simulink model "ASM_Traffic_new"  (R2024a)
settings: Solver=ode1  StartTime=SIM.tstart.v  StopTime=SIM.tend.v  FixedStep=SIM.StepSize.v  RelTol=1e-3
PostLoadFcn:
  | if any(exist('dsrtsu_mdlpostloadfcn', 'file') ~= 0), dsrtsu_mdlpostloadfcn('Execute', bdroot); end
  | try, asm_mdl_postloadfcn(bdroot, 'UpdateModel', 3600); catch, disp(lasterr); end,
InitFcn:
  | , if any(exist('rtifpga_mdlclblib', 'file') ~= 0), rtifpga_mdlclblib('Init', bdroot); end,
  | , if any(exist('dsmpb_private', 'file') ~= 0), dsmpb_private('dsmpb_mdlclblib', 'Init', bdroot); end,
undefined symbols (not defined in the file): _to_, a0b2, ASM_BrakeHydraulics_DemoSystems, ASM_VehicleDynamics_DemoSystems, b98103fe8ad365046cd0, BrakeCircuit, CPT, Crankshaft, DiscIntNeverNeededParam, dsmsi, FinalDriveAssembly, MDL, ModeSignals, Pos_BrakePedal_Maneuver, rad, RefSignals, s_to_rpm, SIM, SoftECU, Suspension, Tire, Transmission
libraries: ASM_Traffic_lib x135, simulink x100, ASM_Utils_lib x77, ASM_VehicleDynamics_lib x70, ASM_Environment_lib x22, dsmpblib x20, dsmsilib x15, MDLD_Utils_lib x10, ASM_BrakeHydraulics_lib x3
(part 4 of 63)

== system ASM_Traffic_new/Environment/Interface_In ==
  note: Environment Traffic
  In : Inport
  Bus Creator1 : BusCreator  Inputs=1
  Bus Selector1 : BusSelector  OutputSignals=Environment.Plant.Sw_ModelPortBlocks[0Disabled|1Enabled],Environment.Plant.Sw_ModelDeskPlottingInterface[0Disabled|1Enabled],VehicleDynamics.Plant.Angle_SteeringWheel[deg],VehicleDynamics.Plant.Angle_SteeringWheel_dt[deg|s],VehicleDynamics.Plant.Trq_SteeringWheel[Nm],VehicleDynamics.Plant.r_Dyn_Tire[FL;FR;RL;RR][m],VehicleDynamics.Plant.Coef_RollingRes[FL;FR;RL;RR][],VehicleDynamics.Plant.CorneringStiffness[FL;FR;RL;RR][N],VehicleDynamics.Plant.Pos_Vehicle_CoorSys_E[x;y;z][m],VehicleDynamics.Plant.Angle_Vehicle_CoorSys_E[x;y;z][deg],VehicleDynamics.Plant.s_Vehicle[m],VehicleDynamics.Plant.v_x_Vehicle_CoG[km|h],VehicleDynamics.Plant.v_y_Vehicle_CoG[km|h],VehicleDynamics.Plant.RollRate_Vehicle_CoG[deg|s],VehicleDynamics.Plant.YawRate_Vehicle_CoG[deg|s],VehicleDynamics.Plant.a_y_Vehicle_CoG[m|s2],VehicleDynamics.Plant.RotationMatrix_V_to_E[1x9],VehicleDynamics.Plant.Const_r_unloaded_Tire_Mean[m],VehicleDynamics.Plant.Coef_RollingRes_Mean[],DomainControl.DriverAssistance.Control.AEB[0|1],DomainControl.DriverAssistance.Control.FCW[0|1],Driver.Plant.Pos_AccPedal[%],Driver.Plant.Pos_BrakePedal[%],Driver.Plant.Pos_ClutchPedal[%],Drivetrain.Plant.Gear[],Driver.Plant.SelectorLever[-3T|-2P|-1R|0N|1D],Driver.Plant.s_Preview[m],Driver.Plant.Angle_SteeringWheel[deg],Driver.Plant.t_Preview_vRef_Driver[s],Drivetrain.Plant.Type_Engine_1[0Unkown|1Other|2Otto|3Diesel|4Electric],Drivetrain.Plant.Trq_Engine_1[Nm],Drivetrain.Plant.n_Engine_1[rpm],Drivetrain.Plant.Type_Engine_2[0Unkown|1Other|2Otto|3Diesel|4Electric],Drivetrain.Plant.Trq_Engine_2[Nm],Drivetrain.Plant.n_Engine_2[rpm],VehicleDynamics.Plant.m_TotalVehicle[kg],DomainControl.StartSystem.Control.State_StartButton[-2|-1|0|1|2|3],DomainControl.DriverAssistance.Control.ACC_State[1OFF|2Standby|3ON],DomainControl.DriverAssistance.Control.Driver_Override_ACC_Active[0Off|1On],DomainControl.DriverAssistance.Control.Driver_Override_ACC_Reason[0NoOverride|1BrakePedal|2AccPedal],VehicleDynamics.Plant.omega_Wheel[rad|s],VehicleDynamics.Plant.Slip_x_Wheel[],VehicleDynamics.Plant.Pos_CP_FL_CoorSys_E[x;y][m],VehicleDynamics.Plant.Pos_CP_FR_CoorSys_E[x;y][m],VehicleDynamics.Plant.Pos_CP_RL_CoorSys_E[x;y][m],VehicleDynamics.Plant.Pos_CP_RL2_CoorSys_E[x;y][m],VehicleDynamics.Plant.Pos_CP_RR_CoorSys_E[x;y][m],VehicleDynamics.Plant.Pos_CP_RR2_CoorSys_E[x;y][m],VehicleDynamics.Plant.Pos_CP_R2L_CoorSys_E[x;y][m],VehicleDynamics.Plant.Pos_CP_R2L2_CoorSys_E[x;y][m],VehicleDynamics.Plant.Pos_CP_R2R_CoorSys_E[x;y][m],VehicleDynamics.Plant.Pos_CP_R2R2_CoorSys_E[x;y][m],Drivetrain.Plant.Mode_Transmission[1Manual|2Automatic],Drivetrain.Plant.Mode_Drivetrain[1|2|3|4|5],VehicleDynamics.Plant.Sw_MasterBrakeCylinder_Mode[1linear|2physical|3Booster],VehicleDynamics.Plant.Active_CP_VehDyn[],VehicleDynamics.Plant.Pos_CP_Front_CoorSys_E[x;y][m],VehicleDynamics.Plant.Pos_CP_Rear_CoorSys_E[x;y][m]
  ModelSignals : Subsystem
  Pos_CP_FL2_Trailer_CoorSys_E[x;y][m] : Constant  Value=[0;0]
  Pos_CP_FL_Trailer_CoorSys_E[x;y][m] : Constant  Value=[0;0]
  Pos_CP_FR2_Trailer_CoorSys_E[x;y][m] : Constant  Value=[0;0]
  Pos_CP_FR_Trailer_CoorSys_E[x;y][m] : Constant  Value=[0;0]
  Pos_CP_R2L2_Trailer_CoorSys_E[x;y][m] : Constant  Value=[0;0]
  Pos_CP_R2L_Trailer_CoorSys_E[x;y][m] : Constant  Value=[0;0]
  Pos_CP_R2R2_Trailer_CoorSys_E[x;y][m] : Constant  Value=[0;0]
  Pos_CP_R2R_Trailer_CoorSys_E[x;y][m] : Constant  Value=[0;0]
  Pos_CP_RL2_Trailer_CoorSys_E[x;y][m] : Constant  Value=[0;0]
  Pos_CP_RL_Trailer_CoorSys_E[x;y][m] : Constant  Value=[0;0]
  Pos_CP_RR2_Trailer_CoorSys_E[x;y][m] : Constant  Value=[0;0]
  Pos_CP_RR_Trailer_CoorSys_E[x;y][m] : Constant  Value=[0;0]
  Out : Outport  VectorParamsAs1DForOutWhenUnconnected=off
  wires:
  Bus Creator1/1 -> Out/1  "Interface_In"
  ModelSignals/1(Out) -> Bus Creator1/1
  Pos_CP_FL_Trailer_CoorSys_E[x;y][m]/1 -> ModelSignals/57(Pos_CP_FL_Trailer_CoorSys_E[x;y][m])
  Pos_CP_FL2_Trailer_CoorSys_E[x;y][m]/1 -> ModelSignals/58(Pos_CP_FL2_Trailer_CoorSys_E[x;y][m])
  Pos_CP_FR_Trailer_CoorSys_E[x;y][m]/1 -> ModelSignals/59(Pos_CP_FR_Trailer_CoorSys_E[x;y][m])
  Pos_CP_FR2_Trailer_CoorSys_E[x;y][m]/1 -> ModelSignals/60(Pos_CP_FR2_Trailer_CoorSys_E[x;y][m])
  Pos_CP_RL_Trailer_CoorSys_E[x;y][m]/1 -> ModelSignals/61(Pos_CP_RL_Trailer_CoorSys_E[x;y][m])
  Pos_CP_RL2_Trailer_CoorSys_E[x;y][m]/1 -> ModelSignals/62(Pos_CP_RL2_Trailer_CoorSys_E[x;y][m])
  Pos_CP_RR_Trailer_CoorSys_E[x;y][m]/1 -> ModelSignals/63(Pos_CP_RR_Trailer_CoorSys_E[x;y][m])
  Pos_CP_RR2_Trailer_CoorSys_E[x;y][m]/1 -> ModelSignals/64(Pos_CP_RR2_Trailer_CoorSys_E[x;y][m])
  Pos_CP_R2L_Trailer_CoorSys_E[x;y][m]/1 -> ModelSignals/65(Pos_CP_R2L_Trailer_CoorSys_E[x;y][m])
  Pos_CP_R2L2_Trailer_CoorSys_E[x;y][m]/1 -> ModelSignals/66(Pos_CP_R2L2_Trailer_CoorSys_E[x;y][m])
  Pos_CP_R2R_Trailer_CoorSys_E[x;y][m]/1 -> ModelSignals/67(Pos_CP_R2R_Trailer_CoorSys_E[x;y][m])
  Pos_CP_R2R2_Trailer_CoorSys_E[x;y][m]/1 -> ModelSignals/68(Pos_CP_R2R2_Trailer_CoorSys_E[x;y][m])
  Bus Selector1/1 -> ModelSignals/1(Sw_ModelPortBlocks[0Disabled|1Enabled])  "<Sw_ModelPortBlocks[0Disabled|1Enabled]>"
  Bus Selector1/2 -> ModelSignals/2(Sw_ModelDeskPlottingInterface[0Disabled|1Enabled])  "<Sw_ModelDeskPlottingInterface[0Disabled|1Enabled]>"
  Bus Selector1/3 -> ModelSignals/3(Angle_SteeringWheel_SteeringSystem[deg])  "<Angle_SteeringWheel[deg]>"
  Bus Selector1/4 -> ModelSignals/4(Angle_SteeringWheel_dt_SteeringSystem[deg|s])  "<Angle_SteeringWheel_dt[deg|s]>"
  Bus Selector1/5 -> ModelSignals/5(Trq_SteeringWheel_SteeringSystem[Nm])  "<Trq_SteeringWheel[Nm]>"
  Bus Selector1/6 -> ModelSignals/6(r_Dyn_Tire[FL;FR;RL;RR][m])  "<r_Dyn_Tire[FL;FR;RL;RR][m]>"
  Bus Selector1/7 -> ModelSignals/7(Coef_RollingRes[FL;FR;RL;RR][])  "<Coef_RollingRes[FL;FR;RL;RR][]>"
  Bus Selector1/8 -> ModelSignals/8(CorneringStiffness[FL;FR;RL;RR][N])  "<CorneringStiffness[FL;FR;RL;RR][N]>"
  Bus Selector1/9 -> ModelSignals/9(Pos_Vehicle_CoorSys_E[x;y;z][m])  "<Pos_Vehicle_CoorSys_E[x;y;z][m]>"
  Bus Selector1/10 -> ModelSignals/10(Angle_Vehicle_CoorSys_E[x;y;z][deg])  "<Angle_Vehicle_CoorSys_E[x;y;z][deg]>"
  Bus Selector1/11 -> ModelSignals/11(s_Vehicle[m])  "<s_Vehicle[m]>"
  Bus Selector1/12 -> ModelSignals/12(v_x_Vehicle_CoG[km|h])  "<v_x_Vehicle_CoG[km|h]>"
  Bus Selector1/13 -> ModelSignals/13(v_y_Vehicle_CoG[km|h])  "<v_y_Vehicle_CoG[km|h]>"
  Bus Selector1/14 -> ModelSignals/14(RollRate_Vehicle_CoG[deg|s])  "<RollRate_Vehicle_CoG[deg|s]>"
  Bus Selector1/15 -> ModelSignals/15(YawRate_Vehicle_CoG[deg|s])  "<YawRate_Vehicle_CoG[deg|s]>"
  Bus Selector1/16 -> ModelSignals/16(a_y_Vehicle_CoG[m|s2])  "<a_y_Vehicle_CoG[m|s2]>"
  Bus Selector1/17 -> ModelSignals/17(RotationMatrix_V_to_E[1x9])  "<RotationMatrix_V_to_E[1x9]>"
  Bus Selector1/18 -> ModelSignals/18(Const_r_unloaded_Tire_Mean[m])  "<Const_r_unloaded_Tire_Mean[m]>"
  Bus Selector1/19 -> ModelSignals/19(Coef_RollingRes_Mean[])  "<Coef_RollingRes_Mean[]>"
  Bus Selector1/20 -> ModelSignals/20(AEB[0|1])  "<AEB[0|1]>"
  Bus Selector1/21 -> ModelSignals/21(FCW[0|1])  "<FCW[0|1]>"
  Bus Selector1/22 -> ModelSignals/22(Pos_AccPedal[%])  "<Pos_AccPedal[%]>"
  Bus Selector1/23 -> ModelSignals/23(Pos_BrakePedal[%])  "<Pos_BrakePedal[%]>"
  Bus Selector1/24 -> ModelSignals/24(Pos_ClutchPedal[%])  "<Pos_ClutchPedal[%]>"
  Bus Selector1/25 -> ModelSignals/25(Gear[])  "<Gear[]>"
  Bus Selector1/26 -> ModelSignals/26(SelectorLever[-3T|-2P|-1R|0N|1D])  "<SelectorLever[-3T|-2P|-1R|0N|1D]>"
  Bus Selector1/27 -> ModelSignals/27(s_Preview[m])  "<s_Preview[m]>"
  Bus Selector1/28 -> ModelSignals/28(Angle_SteeringWheel[deg])  "<Angle_SteeringWheel[deg]>"
  Bus Selector1/29 -> ModelSignals/29(t_Preview_vRef_Driver[s])  "<t_Preview_vRef_Driver[s]>"
  Bus Selector1/30 -> ModelSignals/30(Type_Engine_1[0Unkown|1Other|2Otto|3Diesel|4Electric])  "<Type_Engine_1[0Unkown|1Other|2Otto|3Diesel|4Electric]>"
  Bus Selector1/31 -> ModelSignals/31(Trq_Engine_1[Nm])  "<Trq_Engine_1[Nm]>"
  Bus Selector1/32 -> ModelSignals/32(n_Engine_1[rpm])  "<n_Engine_1[rpm]>"
  Bus Selector1/33 -> ModelSignals/33(Type_Engine_2[0Unkown|1Other|2Otto|3Diesel|4Electric])  "<Type_Engine_2[0Unkown|1Other|2Otto|3Diesel|4Electric]>"
  Bus Selector1/34 -> ModelSignals/34(Trq_Engine_2[Nm])  "<Trq_Engine_2[Nm]>"
  Bus Selector1/35 -> ModelSignals/35(n_Engine_2[rpm])  "<n_Engine_2[rpm]>"
  Bus Selector1/36 -> ModelSignals/36(m_TotalVehicle[kg])  "<m_TotalVehicle[kg]>"
  Bus Selector1/37 -> ModelSignals/37(State_StartButton[-2|-1|0|1|2|3])  "<State_StartButton[-2|-1|0|1|2|3]>"
  Bus Selector1/38 -> ModelSignals/38(ACC_State[1OFF|2Standby|3ON])  "<ACC_State[1OFF|2Standby|3ON]>"
  Bus Selector1/39 -> ModelSignals/39(Driver_Override_ACC_Active[0Off|1On])  "<Driver_Override_ACC_Active[0Off|1On]>"
  Bus Selector1/40 -> ModelSignals/40(Driver_Override_ACC_Reason[0NoOverride|1BrakePedal|2AccPedal])  "<Driver_Override_ACC_Reason[0NoOverride|1BrakePedal|2AccPedal]>"
  Bus Selector1/41 -> ModelSignals/41(omega_Wheel[rad|s])  "<omega_Wheel[rad|s]>"
  Bus Selector1/42 -> ModelSignals/42(Slip_x_Wheel[])  "<Slip_x_Wheel[]>"
  Bus Selector1/43 -> ModelSignals/43(Pos_CP_FL_CoorSys_E[x;y][m])  "<Pos_CP_FL_CoorSys_E[x;y][m]>"
  Bus Selector1/44 -> ModelSignals/44(Pos_CP_FR_CoorSys_E[x;y][m])  "<Pos_CP_FR_CoorSys_E[x;y][m]>"
  Bus Selector1/45 -> ModelSignals/45(Pos_CP_RL_CoorSys_E[x;y][m])  "<Pos_CP_RL_CoorSys_E[x;y][m]>"
  Bus Selector1/46 -> ModelSignals/46(Pos_CP_RL2_CoorSys_E[x;y][m])  "<Pos_CP_RL2_CoorSys_E[x;y][m]>"
  Bus Selector1/47 -> ModelSignals/47(Pos_CP_RR_CoorSys_E[x;y][m])  "<Pos_CP_RR_CoorSys_E[x;y][m]>"
  Bus Selector1/48 -> ModelSignals/48(Pos_CP_RR2_CoorSys_E[x;y][m])  "<Pos_CP_RR2_CoorSys_E[x;y][m]>"
  Bus Selector1/49 -> ModelSignals/49(Pos_CP_R2L_CoorSys_E[x;y][m])  "<Pos_CP_R2L_CoorSys_E[x;y][m]>"
  Bus Selector1/50 -> ModelSignals/50(Pos_CP_R2L2_CoorSys_E[x;y][m])  "<Pos_CP_R2L2_CoorSys_E[x;y][m]>"
  Bus Selector1/51 -> ModelSignals/51(Pos_CP_R2R_CoorSys_E[x;y][m])  "<Pos_CP_R2R_CoorSys_E[x;y][m]>"
  Bus Selector1/52 -> ModelSignals/52(Pos_CP_R2R2_CoorSys_E[x;y][m])  "<Pos_CP_R2R2_CoorSys_E[x;y][m]>"
  Bus Selector1/53 -> ModelSignals/53(Mode_Transmission[1Manual|2Automatic])  "<Mode_Transmission[1Manual|2Automatic]>"
  Bus Selector1/54 -> ModelSignals/54(Mode_Drivetrain[1|2|3|4|5])  "<Mode_Drivetrain[1|2|3|4|5]>"
  Bus Selector1/55 -> ModelSignals/55(Sw_MasterBrakeCylinder_Mode[1linear|2physical|3Booster])  "<Sw_MasterBrakeCylinder_Mode[1linear|2physical|3Booster]>"
  Bus Selector1/56 -> ModelSignals/56(Active_CP_VehDyn_Trailer[])  "<Active_CP_VehDyn[]>"
  Bus Selector1/57 -> ModelSignals/69(Pos_CP_Front_CoorSys_E[x;y][m])  "<Pos_CP_Front_CoorSys_E[x;y][m]>"
  Bus Selector1/58 -> ModelSignals/70(Pos_CP_Rear_CoorSys_E[x;y][m])  "<Pos_CP_Rear_CoorSys_E[x;y][m]>"
  In/1 -> Bus Selector1/1

== system ASM_Traffic_new/Environment/Interface_Out ==
  note: Environment Traffic
  In : Inport
  Activate_DCLink[0Off|1On] : Constant  Value=0
  Animation : Subsystem
  Bus Creator1 : BusCreator  Inputs=2
  Bus Selector1 : BusSelector  OutputSignals=FellowVehicleLights,FellowVehicleDoors  OutputAsBus=on
  Bus Selector{10..12,14,16..18} (7 alike) : BusSelector  OutputSignals=Parameters.Pos_Sensor_Apex_CoorSys_V[x;y;z][m],Parameters.Angle_z_Orientation_Sensor_CoorSys_V[deg],SensorOutput.Angle_Hor_Rel[deg],SensorOutput.Distance[m],Parameters.Num_SensorRays_Used[],Parameters.Angle_ScopeZone_Horizontal[deg]  OutputAsBus=on
  Bus Selector13 : BusSelector  OutputSignals=Line_Sensor_1.Pos_Road_Lane_Animation_CoorSys_E,Line_Sensor_1.Pos_Road_Shape_Line_Animation_CoorSys_E,Line_Sensor_1.Pos_Road_Shape_ContObj_Animation_CoorSys_E,Line_Sensor_1.Pos_Junction_Border_Animation_CoorSys_E,Line_Sensor_1.Pos_Junction_Shape_Line_Animation_CoorSys_E,Line_Sensor_1.Pos_Junction_Shape_ContObj_Animation_CoorSys_E  OutputAsBus=on
  Bus Selector19 : BusSelector  OutputSignals=Sensor_Front_1.SensorOutput[].Traffic_Sign_Valid[0|1],Sensor_Front_1.SensorOutput[].Pos_CoorSys_E[x;y;z][m]  OutputAsBus=on
  Bus Selector20 : BusSelector  OutputSignals=SensorOutput.Pos_Object_NearestPnt_E[x;y;z][m],Info.Flag_Object_In_Scope[0Out|1In],SensorOutput.Flag_NearestPnt_Occluded[-1|0|1]  OutputAsBus=on
  Bus Selector21 : BusSelector  OutputSignals=SensorOutput.Pos_Object_NearestPnt_E[x;y;z][m],Info.Flag_Object_In_Scope[0Out|1In],SensorOutput.Flag_NearestPnt_Occluded[-1|0|1]  OutputAsBus=on
  Bus Selector22 : BusSelector  OutputSignals=ID[],Pos_ObjectPoint_CoorSys_E[x;y;z][m]  OutputAsBus=on
  Bus Selector23 : BusSelector  OutputSignals=ID[],Pos_CoorSys_E[x;y;z][m]  OutputAsBus=on
  Bus Selector24 : BusSelector  OutputSignals=ID[],Pos_ObjectPoint_CoorSys_E[x;y;z][m]  OutputAsBus=on
  Bus Selector25 : BusSelector  OutputSignals=ID[],Pos_ObjectPoint_CoorSys_E[x;y;z][m]  OutputAsBus=on
  Bus Selector26 : BusSelector  OutputSignals=ID[],Pos_CoorSys_E[x;y;z][m]  OutputAsBus=on
  Bus Selector27 : BusSelector  OutputSignals=ID[],Pos_CoorSys_E[x;y;z][m]  OutputAsBus=on
  Bus Selector28 : BusSelector  OutputSignals=SensorOutput.Pos_Object_NearestPnt_E[x;y;z][m],Info.Flag_Object_In_Scope[0Out|1In],SensorOutput.Flag_NearestPnt_Occluded[-1|0|1]  OutputAsBus=on
  Bus Selector3 : BusSelector  OutputSignals=Maneuver.UserInterface.Enable_External_Interfaces.Sw_AnimationInterface[0Disabled|1Enabled],Road.Plant.Road_ASMVeh.s_Veh_Road[m],Road.Plant.LaneSensor_Dynamic.Sensor_Output.CurrentLane.LeftSide.Pos_Left[x;y;z][m],Road.Plant.LaneSensor_Dynamic.Sensor_Output.CurrentLane.LeftSide.Yaw_Angle_Left[deg],Road.Plant.LaneSensor_Dynamic.Sensor_Output.CurrentLane.LeftSide.MarkerType_Left[],Road.Plant.LaneSensor_Dynamic.Sensor_Output.CurrentLane.RightSide.Pos_Right[x;y;z][m],Road.Plant.LaneSensor_Dynamic.Sensor_Output.CurrentLane.RightSide.Yaw_Angle_Right[deg],Road.Plant.LaneSensor_Dynamic.Sensor_Output.Lanes_Right.MarkerType_Right[],Road.Plant.Road_Info.Network_Item_Type_Veh[],Road.Plant.LaneSensor_Dynamic.Sensor_Output.Measurement_Points.Distance_MeasPnt_Marker_Left[m],Road.Plant.LaneSensor_Dynamic.Sensor_Output.Measurement_Points.Distance_MeasPnt_Marker_Right[m],Road.Plant.LaneSensor_Dynamic.Sensor_Output.Measurement_Points.Velocity_MeasPnt_Marker_Left[m|s],Road.Plant.LaneSensor_Dynamic.Sensor_Output.Measurement_Points.Velocity_MeasPnt_Marker_Right[m|s],Road.UserInterface.Objects_DataStreams[],Maneuver.Plant.ManeuverScheduler.Info.ManeuverTime[s],Maneuver.Plant.ManeuverScheduler.Info.ManeuverState[],Maneuver.UserInterface.ManualControl.VehicleLights.Sw_ManualControl_Lights[1Maneuver|2Manual],Maneuver.UserInterface.ManualControl.VehicleLights.Sw_BrakeLight[0Off|1On],Maneuver.UserInterface.ManualControl.VehicleLights.Sw_TurnLights[0Off|1Left|2Right|3Both],Maneuver.Plant.UserSignals_Customized.ASM_Vehicle_TurnLights[],Traffic.Plant.Traffic_Signals_toEnvironment.Pos_Fellows_MainPnt_CoorSys_E[x;y;z][m],Traffic.Plant.Traffic_Signals_toEnvironment.Angle_Fellows[x;y;z][deg],Traffic.Plant.Traffic_Signals_toEnvironment.Flag_FellowUsed[0|1],Traffic.Plant.Traffic_Signals_toEnvironment.v_Fellows_Ref_Scheduler[km|h],Traffic.Plant.Traffic_Signals_toEnvironment.a_Fellows_Ref_Scheduler[m|s2],Traffic.Plant.Traffic_Signals_toEnvironment.v_Fellows[km|h],Traffic.Plant.Traffic_Signals_toEnvironment.UserSignals_Customized,Traffic.UserInterface,Sensors.Plant.Object_Sensor_3D.Boundingboxes_DetectedObjects,Sensors.Plant.Object_Sensor_3D.Sensor_1_Front_Long,Sensors.Plant.Object_Sensor_3D.Sensor_2_Front_Mid,Sensors.Plant.Object_Sensor_3D.Sensor_3_Rear,Sensors.Plant.Object_Sensor_2D.Sensor_1_Front,Sensors.Plant.Object_Sensor_2D.Sensor_2_Front_Left,Sensors.Plant.Object_Sensor_2D.Sensor_3_Left,Sensors.Plant.Object_Sensor_2D.Sensor_4_Rear_Left,Sensors.Plant.Object_Sensor_2D.Sensor_5_Front_Right,Sensors.Plant.Object_Sensor_2D.Sensor_6_Right,Sensors.Plant.Object_Sensor_2D.Sensor_7_Rear_Right,Sensors.Plant.TrafficSign_Sensor_Dyn,Sensors.Plant.Line_Sensor,Sensors.Plant.Object_Sensor_3D.Sensor_1_Front_Long.RadarEffects,Sensors.Plant.Object_Sensor_3D.Sensor_2_Front_Mid.RadarEffects,Sensors.Plant.Object_Sensor_3D.Sensor_3_Rear.RadarEffects,Sensors.Plant.Object_Sensor_3D.Sensor_1_Front_Long.CustomPoints,Sensors.Plant.Object_Sensor_3D.Sensor_2_Front_Mid.CustomPoints,Sensors.Plant.Object_Sensor_3D.Sensor_3_Rear.CustomPoints,Maneuver.Plant.UserSignals_Customized.Mnv_DoorFL[],Maneuver.Plant.UserSignals_Customized.Mnv_DoorFR[],Maneuver.Plant.UserSignals_Customized.Mnv_DoorRL[],Maneuver.Plant.UserSignals_Customized.Mnv_DoorRR[],Maneuver.Plant.UserSignals_Customized.Mnv_Hood[],Maneuver.Plant.UserSignals_Customized.Mnv_Trunk[],Maneuver.UserInterface.ManualControl.Doors.Sw_ManualControl_Doors[1Maneuver|2Manual],Maneuver.UserInterface.ManualControl.Doors.Sw_DoorFL[0Closed_1Open],Maneuver.UserInterface.ManualControl.Doors.Sw_DoorFR[0Closed_1Open],Maneuver.UserInterface.ManualControl.Doors.Sw_DoorRL[0Closed_1Open],Maneuver.UserInterface.ManualControl.Doors.Sw_DoorRR[0Closed_1Open],Maneuver.UserInterface.ManualControl.Doors.Sw_Hood[0Closed_1Open],Maneuver.UserInterface.ManualControl.Doors.Sw_Trunk[0Closed_1Open]
  Bus Selector8 : BusSelector  OutputSignals=Maneuver.Plant.ManeuverScheduler.RefSignals.Pos_AccPedal_Maneuver[%],Maneuver.Plant.ManeuverScheduler.RefSignals.Pos_BrakePedal_Maneuver[%],Maneuver.Plant.ManeuverScheduler.RefSignals.Pos_ClutchPedal_Maneuver[%],Maneuver.Plant.ManeuverScheduler.RefSignals.Gear_Maneuver[],Maneuver.Plant.ManeuverScheduler.RefSignals.Angle_SteeringWheel_Maneuver[deg],Maneuver.Plant.ManeuverScheduler.RefSignals.SelectorLever_Maneuver[],Maneuver.Plant.Sw_TipShift[-1Down|0Off|1Up],Maneuver.Plant.Testbench.n_Engine_Set[rpm],Maneuver.Plant.Testbench.EngOpNum[],Maneuver.Plant.StartButton.Sw_StartButton[0Off|1On],Maneuver.Plant.ManeuverScheduler.RefSignals.v_Vehicle_Ref_Maneuver[m|s],Maneuver.Plant.ManeuverScheduler.RefSignals.v_Vehicle_Ref_Preview_Maneuver[m|s],Maneuver.Plant.ParkingBrake.Sw_ParkingBrake[0Off|1On],Maneuver.Plant.ManeuverScheduler.Parameters.a_x_Max[m|s2],Maneuver.Plant.ManeuverScheduler.Parameters.a_x_Brake_Threshold[m|s2],Maneuver.Plant.ManeuverScheduler.Parameters.a_y_Max[m|s2],Maneuver.Plant.ManeuverScheduler.Parameters.Gear_Max[],Maneuver.Plant.VehicleInitStates.Enable_v_Init[0|1],Traffic.Plant.Traffic_Signals_toEnvironment.a_x_Vehicle_Ref[m|s2],Maneuver.Plant.ManeuverScheduler.Parameters.Width_Deadzone_LatCtrl[m],Road.Plant.Road_ASMVeh.Pos_x_Ref_Veh_Road[m],Road.Plant.Road_ASMVeh.Pos_y_Ref_Veh_Road[m],Maneuver.Plant.ManeuverScheduler.MdlControl.Reset_VehicleStates[0|1],Maneuver.Plant.UserSignals_Customized.ECU_Commands[],Maneuver.Plant.VehicleInitStates.q_dt_Vehicle_Init[6x1],Maneuver.Plant.ManeuverScheduler.RefSignals.Trq_Steering_Maneuver[Nm],Maneuver.Plant.ManeuverScheduler.RefSignals.Sw_SteeringMode_Maneuver[1Angle|2Trq],Maneuver.Plant.ManeuverScheduler.InitialVehStates.s_Vehicle_Init[m],Maneuver.Plant.ManeuverScheduler.InitialVehStates.Route_Direction_Init[],Maneuver.Plant.StartButton.State_StartButton[-1PowerOff|0Acc|1PowerOn|2StarterOn],Road.Plant.Ambient.T_Ambient[degC],Road.Plant.Ambient.p_Ambient[Pa],Road.Plant.Road_ContactPoints.Pos_z_CP[:][m],Road.Plant.Road_ContactPoints.Fric_Coeff_CP[:][],Road.Plant.Road_ContactPoints.UnitVec_z_CP[:][x;y;z],Road.Plant.Road_Init.Pos_Vehicle_Init_CoorSys_E[x;y;z][m],Road.Plant.Road_Init.Angle_Vehicle_Init_CoorSys_E[x;y;z][rad],Road.Plant.Road_ASMVeh.v_Wind_Coor_Sys_E[x;y;z][m|s],Road.Plant.Road_ASMVeh.Slope_Veh_Road[%],Road.Plant.Road_ASMVeh.s_Veh_Road[m],Road.Plant.Road_ASMVeh.s_Total_Veh_Road[m],Road.Plant.Road_ASMVeh.d_Total_Veh_Road[m],Road.Plant.Road_Preview.Curv_Preview_Road[1|m],Road.Plant.Road_Preview.Speed_Limit_Preview_Road[km|h],Road.Plant.Road_Preview.Pos_z_Preview_Road[m],Road.Plant.Road_Preview.Roll_Preview_Road[deg],Road.Plant.Road_Preview.Pitch_Preview_Road[deg],Road.Plant.Road_Preview.x_Preview_DriverCurv[m],Road.Plant.Road_Preview.y_Preview_DriverCurv[m],Road.Plant.Road_Preview.Pos_x_Preview_Road[m],Road.Plant.Road_Preview.Pos_y_Preview_Road[m],Road.Plant.Road_Info.Dist_Border_Left[m],Road.Plant.Road_Info.Dist_Border_Right[m],Road.Plant.Road_ASMVeh.Curv_Veh_Road[1|m],Road.Plant.Road_ASMVeh.Angle_Yaw_Veh_Road[deg],Sensors.Plant.Object_Sensor_3D.Sensor_1_Front_Long.SensorOutput.Dist_Object[m],Sensors.Plant.Object_Sensor_3D.Sensor_1_Front_Long.SensorOutput.v_Rel_Object[m|s],Sensors.Plant.Object_Sensor_3D.Sensor_1_Front_Long.SensorOutput.Angle_Hor_Object[deg],Sensors.Plant.Object_Sensor_3D.Sensor_2_Front_Mid.SensorOutput.Object_ID[],Traffic.Plant.Traffic_Signals_toEnvironment.s_Fellows_Ref_Scheduler[m],Traffic.Plant.FellowSignalLabels.d_Total_Fellows[m],Traffic.Plant.ObjectParameters.FellowParameters.PosVec_MainPnt_Fellows[x;y;z][m],Traffic.Plant.ObjectParameters.FellowParameters.Length_Fellows[m],Traffic.Plant.ObjectParameters.FellowParameters.Width_Fellows[m],Traffic.Plant.ObjectParameters.FellowParameters.Height_Fellows[m],Maneuver.Plant.Testbench.Sw_Testbench[0Off|1On],Maneuver.Plant.ManeuverScheduler.ModeSignals.Mode_AccBr[1Stim|2Driver],Maneuver.Plant.ManeuverScheduler.ModeSignals.Mode_GearClutch[1Stim|2Driver|3OpenClutch|4RefGear],Maneuver.Plant.ManeuverScheduler.ModeSignals.Mode_Steer[1Stim|2Driver|3Fix],Maneuver.Plant.ManeuverScheduler.ModeSignals.Mode_Road[1NoRoad|2Straight|3Circle|4Road],Maneuver.Plant.ManeuverScheduler.ModeSignals.LatDriver[1LatCtrl1|2LatCtrl2],Maneuver.Plant.ManeuverScheduler.ModeSignals.Mode_LatCtrl[1Pos|2Yaw],Maneuver.Plant.ManeuverScheduler.ModeSignals.Mode_AdaptVelocityToRoad[1Off|2On],Maneuver.Plant.ManeuverScheduler.ModeSignals.Mode_ForceToRoad[1Off|2On],Maneuver.Plant.ManeuverScheduler.ModeSignals.Mode_SelectorLever[1Stim|2Driver],Maneuver.Plant.ManeuverScheduler.ModeSignals.Mode_CurvatureCalculation[1Road|2Driver],Maneuver.Plant.ManeuverScheduler.ModeSignals.Mode_TrafficDriver[1Off|2On],Maneuver.Plant.ManeuverScheduler.ModeSignals.Mode_RelativeLane[0CenterLane|1PreferredLane],Maneuver.Plant.StartButton.Mode_StartButtonState[1Stim|2SoftECU],Maneuver.UserInterface.ManualControl.Steering.Sw_Steering_Mode[1Manual|2ManSched],Maneuver.UserInterface.ManualControl.Steering.Const_Steering_Mode_Manual[1Angle|2Trq],Maneuver.Plant.ManeuverScheduler.MdlControl.Keep_VehiclePosition[0|1],Road.Plant.Road_ContactPoints.Sw_Tire_Parameter_Set_CP[:][1|2|3|4],Maneuver.UserInterface.Enable_External_Interfaces.Sw_ModelDeskPlottingInterface[0Disabled|1Enabled],Maneuver.UserInterface.Enable_External_Interfaces.Sw_ModelPortBlocks[0Disabled|1Enabled],Road.Plant.Road_ASMVeh.LaneIdx_Total_Veh_Road[]
  I_Load_HV[A] : Constant  Value=0
  I_Load_LV[A] : Constant  Value=0
  Plant_ModelSignals : Subsystem
  Out : Outport  VectorParamsAs1DForOutWhenUnconnected=off
  wires:
  Bus Selector8/86 -> Plant_ModelSignals/86(Lane_ID_Vehicle[])  "<LaneIdx_Total_Veh_Road[]>"
  Bus Selector3/1 -> Animation/1(Sw_AnimationInterface[0Disabled|1Enabled])  "<Sw_AnimationInterface[0Disabled|1Enabled]>"
  Bus Selector8/85 -> Plant_ModelSignals/85(Sw_ModelPortBlocks[0Disabled|1Enabled])  "<Sw_ModelPortBlocks[0Disabled|1Enabled]>"
  Bus Selector8/84 -> Plant_ModelSignals/84(Sw_ModelDeskPlottingInterface[0Disabled|1Enabled])  "<Sw_ModelDeskPlottingInterface[0Disabled|1Enabled]>"
  Bus Selector3/25 -> Animation/25(a_Fellows_Ref_Scheduler[m|s2])  "<a_Fellows_Ref_Scheduler[m|s2]>"
  Bus Selector11/1 -> Animation/37(ObjectSensor2D_5)
  Bus Selector10/1 -> Animation/36(ObjectSensor2D_4)
  Bus Selector28/1 -> Animation/32(ObjectSensor3D_3)
  Bus Selector16/1 -> Animation/34(ObjectSensor2D_2)
  Bus Selector17/1 -> Animation/35(ObjectSensor2D_3)
  Bus Selector14/1 -> Animation/38(ObjectSensor2D_6)
  Bus Selector18/1 -> Animation/39(ObjectSensor2D_7)
  Bus Selector12/1 -> Animation/33(ObjectSensor2D_1)
  Bus Selector13/1 -> Animation/41(Line_Sensor)
  Bus Selector20/1 -> Animation/30(ObjectSensor3D_1)
  Bus Selector24/1 -> Animation/43(ObjectSensor3D_2_RadarEffects)
  Bus Selector25/1 -> Animation/44(ObjectSensor3D_3_RadarEffects)
  Bus Selector19/1 -> Animation/40(TrafficSign_Sensor_Dyn)
  Bus Selector23/1 -> Animation/45(ObjectSensor3D_1_CustomPoints)
  Bus Selector26/1 -> Animation/46(ObjectSensor3D_2_CustomPoints)
  Bus Selector21/1 -> Animation/31(ObjectSensor3D_2)
  Bus Selector22/1 -> Animation/42(ObjectSensor3D_1_RadarEffects)
  Bus Selector27/1 -> Animation/47(ObjectSensor3D_3_CustomPoints)
  In/1 -> Bus Selector3/1, Bus Selector8/1
  Bus Selector3/14 -> Animation/14(Objects_DataStreams[])  "<Objects_DataStreams[]>"
  Bus Selector3/13 -> Animation/13(Velocity_MeasPnt_Marker_Right[m|s])  "<Velocity_MeasPnt_Marker_Right[m|s]>"
  Bus Selector3/12 -> Animation/12(Velocity_MeasPnt_Marker_Left[m|s])  "<Velocity_MeasPnt_Marker_Left[m|s]>"
  Bus Selector3/11 -> Animation/11(Distance_MeasPnt_Marker_Right[m])  "<Distance_MeasPnt_Marker_Right[m]>"
  Bus Selector3/10 -> Animation/10(Distance_MeasPnt_Marker_Left[m])  "<Distance_MeasPnt_Marker_Left[m]>"
  Bus Selector3/9 -> Animation/9(Network_Item_Type_Veh[])  "<Network_Item_Type_Veh[]>"
  Bus Selector3/8 -> Animation/8(MarkerType_Right[])  "<MarkerType_Right[]>"
  Bus Selector3/7 -> Animation/7(Yaw_Angle_Right[deg])  "<Yaw_Angle_Right[deg]>"
  Bus Selector3/6 -> Animation/6(Pos_Right[x;y;z][m])  "<Pos_Right[x;y;z][m]>"
  Bus Selector3/5 -> Animation/5(MarkerType_Left[])  "<MarkerType_Left[]>"
  Bus Selector3/4 -> Animation/4(Yaw_Angle_Left[deg])  "<Yaw_Angle_Left[deg]>"
  Bus Selector3/3 -> Animation/3(Pos_Left[x;y;z][m])  "<Pos_Left[x;y;z][m]>"
  Bus Selector3/2 -> Animation/2(s_Veh_Road[m])  "<s_Veh_Road[m]>"
  Bus Selector8/18 -> Plant_ModelSignals/18(Enable_v_Init[0|1])  "<Enable_v_Init[0|1]>"
  Bus Selector8/30 -> Plant_ModelSignals/30(State_StartButton[-1PowerOff|0Acc|1PowerOn|2StarterOn])  "<State_StartButton[-1PowerOff|0Acc|1PowerOn|2StarterOn]>"
  Bus Selector8/29 -> Plant_ModelSignals/29(Route_Direction_Init[])  "<Route_Direction_Init[]>"
  Bus Selector8/28 -> Plant_ModelSignals/28(s_Vehicle_Init[m])  "<s_Vehicle_Init[m]>"
  Bus Selector8/27 -> Plant_ModelSignals/27(Sw_SteeringMode[1Angle|2Trq])  "<Sw_SteeringMode_Maneuver[1Angle|2Trq]>"
  Bus Selector8/26 -> Plant_ModelSignals/26(Trq_Driver_External[Nm])  "<Trq_Steering_Maneuver[Nm]>"
  Bus Selector8/25 -> Plant_ModelSignals/25(q_dt_Vehicle_Init[6x1])  "<q_dt_Vehicle_Init[6x1]>"
  Bus Selector8/24 -> Plant_ModelSignals/24(ECU_Commands[])  "<ECU_Commands[]>"
  Bus Selector8/23 -> Plant_ModelSignals/23(Reset_VehicleStates[0|1])  "<Reset_VehicleStates[0|1]>"
  Bus Selector8/22 -> Plant_ModelSignals/22(Pos_y_Ref_Vehicle_Road[m])  "<Pos_y_Ref_Veh_Road[m]>"
  Bus Selector8/21 -> Plant_ModelSignals/21(Pos_x_Ref_Vehicle_Road[m])  "<Pos_x_Ref_Veh_Road[m]>"
  Bus Selector8/20 -> Plant_ModelSignals/20(Width_Deadzone_LatCtrl[m])  "<Width_Deadzone_LatCtrl[m]>"
  Bus Selector8/19 -> Plant_ModelSignals/19(a_x_Vehicle_Ref_TrafficDriver[m|s2])  "<a_x_Vehicle_Ref[m|s2]>"
  Bus Selector8/17 -> Plant_ModelSignals/17(Gear_Max[0Off|1_n])  "<Gear_Max[]>"
  Bus Selector8/16 -> Plant_ModelSignals/16(a_y_Max[m|s2])  "<a_y_Max[m|s2]>"
  Bus Selector8/15 -> Plant_ModelSignals/15(a_x_Min[m|s2])  "<a_x_Brake_Threshold[m|s2]>"
  Bus Selector8/14 -> Plant_ModelSignals/14(a_x_Max[m|s2])  "<a_x_Max[m|s2]>"
  Bus Selector8/13 -> Plant_ModelSignals/13(Sw_ParkingBrake[0Off|1On])  "<Sw_ParkingBrake[0Off|1On]>"
  Bus Selector8/12 -> Plant_ModelSignals/12(v_Vehicle_Preview_Ref_Maneuver[m|s])  "<v_Vehicle_Ref_Preview_Maneuver[m|s]>"
  Bus Selector8/11 -> Plant_ModelSignals/11(v_Vehicle_Ref_Maneuver[m|s])  "<v_Vehicle_Ref_Maneuver[m|s]>"
  Bus Selector8/10 -> Plant_ModelSignals/10(Sw_StartButton[0Off|1On])  "<Sw_StartButton[0Off|1On]>"
  Bus Selector8/9 -> Plant_ModelSignals/9(EngOPNum[])  "<EngOpNum[]>"
  Bus Selector8/8 -> Plant_ModelSignals/8(n_Engine_Set[rpm])  "<n_Engine_Set[rpm]>"
  Bus Selector8/7 -> Plant_ModelSignals/7(Sw_TipShift_Maneuver[-1Down|0Off|1Up])  "<Sw_TipShift[-1Down|0Off|1Up]>"
  Bus Selector8/6 -> Plant_ModelSignals/6(SelectorLever_Maneuver[-3T|-2P|-1R|0N|1D])  "<SelectorLever_Maneuver[]>"
  Bus Selector8/5 -> Plant_ModelSignals/5(Angle_SteeringWheel_Maneuver[deg])  "<Angle_SteeringWheel_Maneuver[deg]>"
  Bus Selector8/4 -> Plant_ModelSignals/4(Gear_Maneuver[])  "<Gear_Maneuver[]>"
  Bus Selector8/3 -> Plant_ModelSignals/3(Pos_ClutchPedal_Maneuver[%])  "<Pos_ClutchPedal_Maneuver[%]>"
  Bus Selector8/2 -> Plant_ModelSignals/2(Pos_BrakePedal_Maneuver[%])  "<Pos_BrakePedal_Maneuver[%]>"
  Bus Selector8/1 -> Plant_ModelSignals/1(Pos_AccPedal_Maneuver[%])  "<Pos_AccPedal_Maneuver[%]>"
  Bus Creator1/1 -> Out/1  "Environment"
  I_Load_LV[A]/1 -> Plant_ModelSignals/89(I_Load_LV[A])
  I_Load_HV[A]/1 -> Plant_ModelSignals/88(I_Load_HV[A])
  Activate_DCLink[0Off|1On]/1 -> Plant_ModelSignals/87(Activate_DCLink[0Off|1On])
  Bus Selector8/83 -> Plant_ModelSignals/83(Sw_Tire_Parameter_Set_CP[:][1|2|3|4])  "<Sw_Tire_Parameter_Set_CP[:][1|2|3|4]>"
  Bus Selector8/82 -> Plant_ModelSignals/82(Keep_VehiclePosition[0|1])  "<Keep_VehiclePosition[0|1]>"
  Bus Selector8/31 -> Plant_ModelSignals/31(T_Ambient[degC])  "<T_Ambient[degC]>"
  Bus Selector8/32 -> Plant_ModelSignals/32(p_Ambient[Pa])  "<p_Ambient[Pa]>"
  Bus Selector8/33 -> Plant_ModelSignals/33(Pos_z_CP[:][m])  "<Pos_z_CP[:][m]>"
  Bus Selector8/34 -> Plant_ModelSignals/34(Fric_Coeff_CP[:][])  "<Fric_Coeff_CP[:][]>"
  Bus Selector8/35 -> Plant_ModelSignals/35(UnitVec_z_CP[:][x;y;z])  "<UnitVec_z_CP[:][x;y;z]>"
  Bus Selector8/36 -> Plant_ModelSignals/36(Pos_Vehicle_Init_CoorSys_E[x;y;z][m])  "<Pos_Vehicle_Init_CoorSys_E[x;y;z][m]>"
  Bus Selector8/37 -> Plant_ModelSignals/37(Angle_Vehicle_Init_CoorSys_E[x;y;z][rad])  "<Angle_Vehicle_Init_CoorSys_E[x;y;z][rad]>"
  Bus Selector8/38 -> Plant_ModelSignals/38(v_Wind_Coor_Sys_E[x;y;z][m|s])  "<v_Wind_Coor_Sys_E[x;y;z][m|s]>"
  Bus Selector8/39 -> Plant_ModelSignals/39(Slope_Veh_Road[%])  "<Slope_Veh_Road[%]>"
  Bus Selector8/40 -> Plant_ModelSignals/40(s_Vehicle_Road[m])  "<s_Veh_Road[m]>"
  Bus Selector8/41 -> Plant_ModelSignals/41(s_Total_Vehicle_Road[m])  "<s_Total_Veh_Road[m]>"
  Bus Selector8/42 -> Plant_ModelSignals/42(d_Vehicle_Road[m])  "<d_Total_Veh_Road[m]>"
  Bus Selector8/43 -> Plant_ModelSignals/43(Curv_Preview_Road[1|m])  "<Curv_Preview_Road[1|m]>"
  Bus Selector8/44 -> Plant_ModelSignals/44(Speed_Limit_Preview_Road[km|h])  "<Speed_Limit_Preview_Road[km|h]>"
  Bus Selector8/45 -> Plant_ModelSignals/45(Pos_z_Preview_Road[m])  "<Pos_z_Preview_Road[m]>"
  Bus Selector8/46 -> Plant_ModelSignals/46(Roll_Preview_Road[deg])  "<Roll_Preview_Road[deg]>"
  Bus Selector8/47 -> Plant_ModelSignals/47(Pitch_Preview_Road[deg])  "<Pitch_Preview_Road[deg]>"
  Bus Selector8/48 -> Plant_ModelSignals/48(x_Preview_DriverCurv[m])  "<x_Preview_DriverCurv[m]>"
  Bus Selector8/49 -> Plant_ModelSignals/49(y_Preview_DriverCurv[m])  "<y_Preview_DriverCurv[m]>"
  Bus Selector8/50 -> Plant_ModelSignals/50(Pos_x_Preview_Road[m])  "<Pos_x_Preview_Road[m]>"
  Bus Selector8/51 -> Plant_ModelSignals/51(Pos_y_Preview_Road[m])  "<Pos_y_Preview_Road[m]>"
  Bus Selector8/52 -> Plant_ModelSignals/52(Dist_Border_Left[m])  "<Dist_Border_Left[m]>"
  Bus Selector8/53 -> Plant_ModelSignals/53(Dist_Border_Right[m])  "<Dist_Border_Right[m]>"
  Bus Selector8/54 -> Plant_ModelSignals/54(Curv_Vehicle_Road[1|m])  "<Curv_Veh_Road[1|m]>"
  Bus Selector8/55 -> Plant_ModelSignals/55(Angle_Yaw_Veh_Road[deg])  "<Angle_Yaw_Veh_Road[deg]>"
  Bus Selector8/56 -> Plant_ModelSignals/56(Dist_Fellows[m])  "<Dist_Object[m]>"
  Bus Selector8/57 -> Plant_ModelSignals/57(v_Rel_Fellows[m|s])  "<v_Rel_Object[m|s]>"
  Bus Selector8/58 -> Plant_ModelSignals/58(Angle_Hor_Rel_Fellows[deg])  "<Angle_Hor_Object[deg]>"
  Bus Selector8/59 -> Plant_ModelSignals/59(Object_ID[])  "<Object_ID[]>"
  Bus Selector8/60 -> Plant_ModelSignals/60(s_Fellows_Ref[m])  "<s_Fellows_Ref_Scheduler[m]>"
  Bus Selector8/61 -> Plant_ModelSignals/61(d_Total_Fellows[m])  "<d_Total_Fellows[m]>"
  Bus Selector8/62 -> Plant_ModelSignals/62(PosVec_MainPnt_Fellows[x;y;z][m])  "<PosVec_MainPnt_Fellows[x;y;z][m]>"
  Bus Selector8/63 -> Plant_ModelSignals/63(Length_Fellows[m])  "<Length_Fellows[m]>"
  Bus Selector8/64 -> Plant_ModelSignals/64(Width_Fellows[m])  "<Width_Fellows[m]>"
  Bus Selector8/65 -> Plant_ModelSignals/65(Height_Fellows[m])  "<Height_Fellows[m]>"
  Bus Selector8/66 -> Plant_ModelSignals/66(Sw_Testbench[0Off|1On])  "<Sw_Testbench[0Off|1On]>"
  Bus Selector8/67 -> Plant_ModelSignals/67(Mode_AcceleratorBrake[1Stim|2Driver])  "<Mode_AccBr[1Stim|2Driver]>"
  Bus Selector8/68 -> Plant_ModelSignals/68(Mode_GearClutch[1Stim|2Driver|3OpenClutch|4RefGear])  "<Mode_GearClutch[1Stim|2Driver|3OpenClutch|4RefGear]>"
  Bus Selector8/69 -> Plant_ModelSignals/69(Mode_Steer[1Stim|2Driver|3Fix])  "<Mode_Steer[1Stim|2Driver|3Fix]>"
  Bus Selector8/70 -> Plant_ModelSignals/70(Mode_Road[1NoRoad|2Straight|3Circle|4Road])  "<Mode_Road[1NoRoad|2Straight|3Circle|4Road]>"
  Bus Selector8/71 -> Plant_ModelSignals/71(Sw_LatDriver[1LatCtrl1|2LatCtrl2])  "<LatDriver[1LatCtrl1|2LatCtrl2]>"
  Bus Selector8/72 -> Plant_ModelSignals/72(Mode_LatCtrl[1Pos|2Yaw])  "<Mode_LatCtrl[1Pos|2Yaw]>"
  Bus Selector8/73 -> Plant_ModelSignals/73(Mode_AdaptVelocityToRoad[1Off|2On])  "<Mode_AdaptVelocityToRoad[1Off|2On]>"
  Bus Selector8/74 -> Plant_ModelSignals/74(Mode_ForceToRoad[1Off|2On])  "<Mode_ForceToRoad[1Off|2On]>"
  Bus Selector8/75 -> Plant_ModelSignals/75(Mode_SelectorLever[1Stim|2Driver])  "<Mode_SelectorLever[1Stim|2Driver]>"
  Bus Selector8/76 -> Plant_ModelSignals/76(Mode_CurvatureCalculation[1Road|2Driver])  "<Mode_CurvatureCalculation[1Road|2Driver]>"
  Bus Selector8/77 -> Plant_ModelSignals/77(Mode_TrafficDriver[1Off|2On])  "<Mode_TrafficDriver[1Off|2On]>"
  Bus Selector8/78 -> Plant_ModelSignals/78(Mode_RelativeLane[0CenterLane|1PreferredLane])  "<Mode_RelativeLane[0CenterLane|1PreferredLane]>"
  Bus Selector8/79 -> Plant_ModelSignals/79(Mode_StartButtonState[1Stim|2SoftECU])  "<Mode_StartButtonState[1Stim|2SoftECU]>"
  Bus Selector8/80 -> Plant_ModelSignals/80(Sw_Steering_Mode[1Manual|2ManSched])  "<Sw_Steering_Mode[1Manual|2ManSched]>"
  Bus Selector8/81 -> Plant_ModelSignals/81(Const_Steering_Mode_Manual[1Angle|2Trq])  "<Const_Steering_Mode_Manual[1Angle|2Trq]>"
  Plant_ModelSignals/1(Out) -> Bus Creator1/1
  Animation/1(Out) -> Bus Creator1/2
  Bus Selector3/47 -> Bus Selector27/1  "<CustomPoints>"
  Bus Selector3/46 -> Bus Selector26/1  "<CustomPoints>"
  Bus Selector3/45 -> Bus Selector23/1  "<CustomPoints>"
  Bus Selector3/44 -> Bus Selector25/1  "<RadarEffects>"
  Bus Selector3/43 -> Bus Selector24/1  "<RadarEffects>"
  Bus Selector3/42 -> Bus Selector22/1  "<RadarEffects>"
  Bus Selector3/41 -> Bus Selector13/1  "<Line_Sensor>"
  Bus Selector3/40 -> Bus Selector19/1  "<TrafficSign_Sensor_Dyn>"
  Bus Selector3/39 -> Bus Selector18/1  "<Sensor_7_Rear_Right>"
  Bus Selector3/38 -> Bus Selector14/1  "<Sensor_6_Right>"
  Bus Selector3/37 -> Bus Selector11/1  "<Sensor_5_Front_Right>"
  Bus Selector3/36 -> Bus Selector10/1  "<Sensor_4_Rear_Left>"
  Bus Selector3/35 -> Bus Selector17/1  "<Sensor_3_Left>"
  Bus Selector3/34 -> Bus Selector16/1  "<Sensor_2_Front_Left>"
  Bus Selector3/33 -> Bus Selector12/1  "<Sensor_1_Front>"
  Bus Selector3/32 -> Bus Selector28/1  "<Sensor_3_Rear>"
  Bus Selector3/31 -> Bus Selector21/1  "<Sensor_2_Front_Mid>"
  Bus Selector3/30 -> Bus Selector20/1  "<Sensor_1_Front_Long>"
  Bus Selector3/15 -> Animation/15(ManeuverTime[s])  "<ManeuverTime[s]>"
  Bus Selector3/16 -> Animation/16(ManeuverState[])  "<ManeuverState[]>"
  Bus Selector3/17 -> Animation/17(Sw_ManualControl_Lights[1Maneuver|2Manual])  "<Sw_ManualControl_Lights[1Maneuver|2Manual]>"
  Bus Selector3/18 -> Animation/18(Sw_BrakeLight[0Off|1On])  "<Sw_BrakeLight[0Off|1On]>"
  Bus Selector3/19 -> Animation/19(Sw_TurnLights[0Off|1Left|2Right|3Both])  "<Sw_TurnLights[0Off|1Left|2Right|3Both]>"
  Bus Selector3/20 -> Animation/20(ASM_Vehicle_TurnLights[])  "<ASM_Vehicle_TurnLights[]>"
  Bus Selector3/21 -> Animation/21(Pos_Fellows_MainPnt_CoorSys_E[x;y;z][m])  "<Pos_Fellows_MainPnt_CoorSys_E[x;y;z][m]>"
  Bus Selector3/22 -> Animation/22(Angle_Fellows[x;y;z][deg])  "<Angle_Fellows[x;y;z][deg]>"
  Bus Selector3/23 -> Animation/23(Flag_FellowUsed[0|1])  "<Flag_FellowUsed[0|1]>"
  Bus Selector3/24 -> Animation/24(v_Fellows_Ref_Scheduler[km|h])  "<v_Fellows_Ref_Scheduler[km|h]>"
  Bus Selector3/26 -> Animation/26(v_Fellows[km|h])  "<v_Fellows[km|h]>"
  Bus Selector3/27 -> Animation/27(UserSignals_Customized)  "<UserSignals_Customized>"
  Bus Selector3/28 -> Bus Selector1/1  "<UserInterface>"
  Bus Selector3/29 -> Animation/29(Boundingbox_DetectedObjects)  "<Boundingboxes_DetectedObjects>"
  Bus Selector1/1 -> Animation/28(Settings)
  Bus Selector3/49 -> Animation/49(Mnv_DoorFR[])  "<Mnv_DoorFR[]>"
  Bus Selector3/50 -> Animation/50(Mnv_DoorRL[])  "<Mnv_DoorRL[]>"
  Bus Selector3/51 -> Animation/51(Mnv_DoorRR[])  "<Mnv_DoorRR[]>"
  Bus Selector3/52 -> Animation/52(Mnv_Hood[])  "<Mnv_Hood[]>"
  Bus Selector3/53 -> Animation/53(Mnv_Trunk[])  "<Mnv_Trunk[]>"
  Bus Selector3/54 -> Animation/54(Sw_ManualControl_Doors[1Maneuver|2Manual])  "<Sw_ManualControl_Doors[1Maneuver|2Manual]>"
  Bus Selector3/55 -> Animation/55(Sw_DoorFL[0Closed_1Open])  "<Sw_DoorFL[0Closed_1Open]>"
  Bus Selector3/56 -> Animation/56(Sw_DoorFR[0Closed_1Open])  "<Sw_DoorFR[0Closed_1Open]>"
  Bus Selector3/57 -> Animation/57(Sw_DoorRL[0Closed_1Open])  "<Sw_DoorRL[0Closed_1Open]>"
  Bus Selector3/58 -> Animation/58(Sw_DoorRR[0Closed_1Open])  "<Sw_DoorRR[0Closed_1Open]>"
  Bus Selector3/59 -> Animation/59(Sw_Hood[0Closed_1Open])  "<Sw_Hood[0Closed_1Open]>"
  Bus Selector3/60 -> Animation/60(Sw_Trunk[0Closed_1Open])  "<Sw_Trunk[0Closed_1Open]>"
  Bus Selector3/48 -> Animation/48(Mnv_DoorFL[])  "<Mnv_DoorFL[]>"

== system ASM_Traffic_new/Environment/Maneuver ==
  note: Maneuver
  In : Inport
  Bus Creator2 : BusCreator  Inputs=2
  PlantModel : Subsystem
  UserInterface : Subsystem
  Out : Outport  VectorParamsAs1DForOutWhenUnconnected=off
  wires:
  Bus Creator2/1 -> Out/1  "Maneuver"
  In/1 -> UserInterface/1(Interface_In), PlantModel/2(In)
  UserInterface/1(Out) -> Bus Creator2/2, PlantModel/1(UserInterface)
  PlantModel/1(ASMSignalBus) -> UserInterface/2(In), Bus Creator2/1

== system ASM_Traffic_new/Environment/Road ==
  note: Road
  In : Inport
  Bus Creator2 : BusCreator  Inputs=2
  PlantModel : Subsystem
  UserInterface : Subsystem
  Out : Outport  VectorParamsAs1DForOutWhenUnconnected=off
  wires:
  In/1 -> UserInterface/1(Interface_In), PlantModel/2(In)
  PlantModel/1(ASMSignalBus) -> UserInterface/2(In), Bus Creator2/1
  UserInterface/1(Out) -> Bus Creator2/2, PlantModel/1(UserInterface)
  Bus Creator2/1 -> Out/1  "Road"

== system ASM_Traffic_new/Environment/Sensors ==
  note: Sensors
  In : Inport
  Bus Creator1 : BusCreator  Inputs=1
  PlantModel : Subsystem
  UserInterface : Subsystem
  Out : Outport  VectorParamsAs1DForOutWhenUnconnected=off
  wires:
  In/1 -> PlantModel/2(In)
  UserInterface/1(Out) -> PlantModel/1(UserInterface)
  Bus Creator1/1 -> Out/1  "Sensors"
  PlantModel/1(ASMSignalBus) -> UserInterface/1(In), Bus Creator1/1

== system ASM_Traffic_new/Environment/SignalInterface ==
  In : Inport
  ASMSignalInterface : Subsystem  mask(ASM_SIGNAL_INTERFACE){LabelTextfield=Environment}
      mask prompts: LabelTextfield "Label"
      mask help:
      | The ASMSignalInterface block processes the ASMSignalBus and provides a vector-based interface for each signal (e.g. ModelDesk Plotting).
      |
      | Always push the update button after you have changed the signal bus structure in order to synchronize the signal interface. The update may take a few seconds.
      | A modified model must be reloaded in ModelDesk to keep consistency of ModelDesk and simulation model plot signals. Therefore select ''Update Model'' from the ''Simulation Model'' context menu of the ModelDesk Project Navigator.
      settings: AttributesFormatString=Label: %<LabelTextfield>
      settings: CopyFcn=|
      | try
      |  set_param(gcb,'LinkStatus', 'none')
      | catch
      | end
      mask Help: eval(['asm_modelhelp(gcbh,''tool'',''ASM_Utils_lib'', ''ASMSIGNALINTERFACE'')'])
      mask DialogControl Hint Prompt: For changes of Label first apply change and then push "Update".
      mask DialogControl UpdateButton Prompt: Update
      mask DialogControl UpdateButton Callback: asm_mdld_plot_block_update(bdroot(gcb), 'update', 'current');
      mask DialogControl UpdateAllButton Prompt: Update All
      mask DialogControl UpdateAllButton Callback: asm_mdld_plot_block_update(bdroot(gcb), 'update', 'all');
  Bus Creator : BusCreator  Inputs=5
  Bus Selector : BusSelector  OutputSignals=ManeuverScheduler,UserSignals_Customized,VehicleInitStates,Testbench,ParkingBrake,StartButton,Sw_TipShift[-1Down|0Off|1Up]  OutputAsBus=on
  Bus Selector1 : BusSelector  OutputSignals=Road_Init,Road_ASMVeh,Road_ContactPoints,Road_Preview,Road_Info,Road_TrafficFellows,UserSignals,TrafficObject_Data[],UserSignals_Customized,Pos_Vehicle_GPS[Long;Lat][deg],Ambient,LaneSensor_Dynamic,Lane_Network  OutputAsBus=on
  Bus Selector2 : BusSelector  OutputSignals=Traffic_Signals_toEnvironment,FellowSignalLabels,ObjectParameters  OutputAsBus=on
  Bus Selector3 : BusSelector  OutputSignals=Object_Sensor_3D,Object_Sensor_2D,TrafficSign_Sensor_Dyn,Line_Sensor,Collision_Sensor,Sensors_Common  OutputAsBus=on
  Bus Selector4 : BusSelector  OutputSignals=Control,Info,Data,Data_Access,OpenSimulationInterface  OutputAsBus=on
  Bus Selector Disable Signals : BusSelector  OutputSignals=Interface_In.ExternalModel.Sw_ModelPortBlocks[0Disabled|1Enabled],Interface_In.ExternalModel.Sw_ModelDeskPlottingInterface[0Disabled|1Enabled]
  ExternalOutports : Subsystem  TreatAsAtomicUnit=on
  Reduce_ASMSignalBus : Subsystem
  wires:
  Bus Selector Disable Signals/2 -> ASMSignalInterface/Enable  "<Sw_ModelDeskPlottingInterface[0Disabled|1Enabled]>"
  Bus Selector Disable Signals/1 -> ExternalOutports/Enable  "<Sw_ModelPortBlocks[0Disabled|1Enabled]>"
  In/1 -> Bus Selector Disable Signals/1
  Bus Selector1/1 -> Bus Creator/2  "Road"
  [ASMBUS_Environment_Maneuver] -> Bus Selector/1
  Bus Selector/1 -> Bus Creator/1  "Maneuver"
  [ASMBUS_Environment_Road] -> Bus Selector1/1
  [ASMBUS_Environment_Traffic_FellowMovement] -> Bus Selector2/1
  Bus Selector2/1 -> Bus Creator/3  "Traffic"
  Bus Selector3/1 -> Bus Creator/4  "Sensors"
  [ASMBUS_Environment_Traffic_Sensors] -> Bus Selector3/1
  Bus Selector4/1 -> Bus Creator/5  "GroundTruth"
  [ASMBUS_Traffic_GroundTruth] -> Bus Selector4/1
  Bus Creator/1 -> Reduce_ASMSignalBus/1(ASMSignalBus), ExternalOutports/1(In1)
  Reduce_ASMSignalBus/1(ASMSignalBus_Reduced) -> ASMSignalInterface/1(ASMSignalBus)

== system ASM_Traffic_new/Environment/Traffic ==
  note: Traffic
  In : Inport
  Bus Creator1 : BusCreator  Inputs=2
  PlantModel : Subsystem
  UserInterface : Subsystem
  Out : Outport  VectorParamsAs1DForOutWhenUnconnected=off
  wires:
  In/1 -> PlantModel/2(In)
  PlantModel/1(ASMSignalBus) -> Bus Creator1/1, UserInterface/1(In)
  Bus Creator1/1 -> Out/1  "Traffic"
  UserInterface/1(Out) -> PlantModel/1(UserInterface), Bus Creator1/2

== system ASM_Traffic_new/VehicleDynamics/Control ==
  note: Vehicle Dynamics Control
  Interface_In : Inport
  Plant : Inport  Port=2
  Bus Creator1 : BusCreator  Inputs=2
  Bus Creator5 : BusCreator  Inputs=2
  SoftECU_Brake : Subsystem
  SoftECU_Steering : Subsystem
  Sw_ECU_Brake_Signals : Subsystem
  Sw_ECU_Steering_Signals : Subsystem
  UserInterface : Subsystem
  Control : Outport  VectorParamsAs1DForOutWhenUnconnected=off
  wires:
  Sw_ECU_Steering_Signals/1(ECU_Signals) -> Bus Creator5/2
  SoftECU_Steering/2(Out) -> Sw_ECU_Steering_Signals/1(SoftECU)
  SoftECU_Brake/2(Out) -> Sw_ECU_Brake_Signals/1(SoftECU)
  Interface_In/1 -> SoftECU_Steering/2(Interface_In), Sw_ECU_Steering_Signals/2(ExternalECU), Sw_ECU_Brake_Signals/2(ExternalECU), SoftECU_Brake/2(Interface_In)
  Sw_ECU_Brake_Signals/1(ECU_Signals) -> Bus Creator5/1
  Bus Creator5/1 -> Control/1  "Control"
  SoftECU_Brake/1(ASMSignalBus) -> Bus Creator1/1
  SoftECU_Steering/1(ASMSignalBus) -> Bus Creator1/2
  Bus Creator1/1 -> UserInterface/1(In)  "Control"
  Plant/1 -> SoftECU_Steering/3(Plant), SoftECU_Brake/3(Plant)
  UserInterface/1(Out) -> SoftECU_Steering/1(UserInterface), SoftECU_Brake/1(UserInterface)
